simulink model "ARIES"  (R2024b)
settings: Solver=ode4  StartTime=0.0  StopTime=8*18601.8746  FixedStep=1e-1  RelTol=1e-3
model workspace (MAT data in the model file):
  BVH_bboxMax : Simulink.Parameter (value not decoded)
  BVH_bboxMin : Simulink.Parameter (value not decoded)
  BVH_fCount : Simulink.Parameter (value not decoded)
  BVH_fStart : Simulink.Parameter (value not decoded)
  BVH_faces : Simulink.Parameter (value not decoded)
  BVH_left : Simulink.Parameter (value not decoded)
  BVH_normals : Simulink.Parameter (value not decoded)
  BVH_right : Simulink.Parameter (value not decoded)
  BVH_vertexList : Simulink.Parameter (value not decoded)
  WP_NWaypoints : Simulink.Parameter (value not decoded)
  WP_STMArcs : Simulink.Parameter (value not decoded)
  WP_burnStrategy : Simulink.Parameter (value not decoded)
  WP_dtArc : Simulink.Parameter (value not decoded)
  WP_proxRadius : Simulink.Parameter (value not decoded)
  WP_waypointPosition : Simulink.Parameter (value not decoded)
  WP_waypointVelocity : Simulink.Parameter (value not decoded)
  asteroidAngularVelocity : Simulink.Parameter (value not decoded)
values from neighbouring files (symbols this model uses):
  actuators = actuatorsConfig()    [mainMontecarlo.m]    (also in mainSimulator.m)
  environment = environmentConfig(gravDataPath)    [mainMontecarlo.m]    (also in mainSimulator.m; mainWaypointGenerator.m = environmentConfig(gravDataPath, true))
  gravAtt = Simulink.Parameter(environment.gravStruct.gravAtt)    [mainSimulator.m]    (also in mainWaypointGenerator.m)
  init = initConditionConfig(control)    [mainMontecarlo.m]    (also in mainSimulator.m)
  simulation = simulationConfig()    [mainMontecarlo.m]    (also in mainSimulator.m = simulationConfig(control, environment))
symbols that are objects in the model workspace (value not decoded): asteroidAngularVelocity, BVH_bboxMax, BVH_bboxMin, BVH_faces, BVH_fCount, BVH_fStart, BVH_left, BVH_right, BVH_vertexList, WP_burnStrategy, WP_dtArc, WP_NWaypoints, WP_proxRadius, WP_STMArcs, WP_waypointPosition, WP_waypointVelocity
undefined symbols (not defined in the file or in its folder): control, magnitude, spacecraft
libraries: matrix_library x14, aerolibutil x4, sharedutil x2, sharedtransform x2, simulink x2
(part 2 of 2)

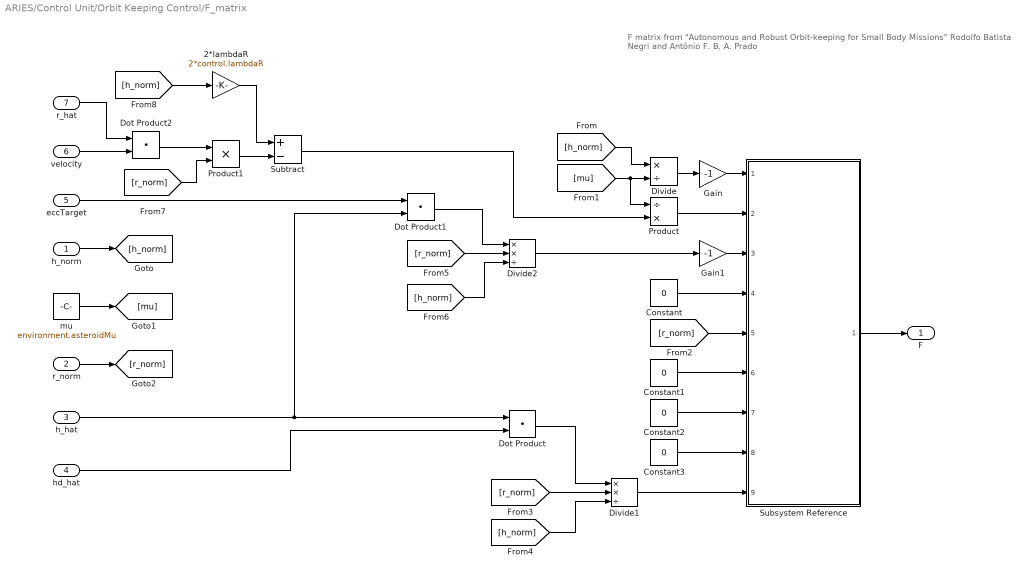
== system ARIES/Control Unit/Orbit Keeping Control/F_matrix ==
  note: F matrix from
      | "Autonomous and Robust Orbit-keeping for Small Body Missions"
      | Rodolfo Batista Negri and Antônio F. B. A. Prado
  h_norm : Inport
  r_norm : Inport  Port=2
  h_hat : Inport  Port=3
  hd_hat : Inport  Port=4
  eccTarget : Inport  Port=5
  velocity : Inport  Port=6
  r_hat : Inport  Port=7
  2*lambdaR : Gain  Gain=2*control.lambdaR
  Constant{,1..3} (4 alike) : Constant  Value=0
  Divide : Product  Inputs=*/
  Divide1 : Product  Inputs=**/
  Divide2 : Product  Inputs=**/
  Dot Product : DotProduct  OutDataTypeStr=Inherit: Inherit via internal rule
  Dot Product1 : DotProduct  OutDataTypeStr=Inherit: Inherit via internal rule
  Dot Product2 : DotProduct  OutDataTypeStr=Inherit: Inherit via internal rule
  Gain : Gain  Gain=-1
  Gain1 : Gain  Gain=-1
  Product : Product  Inputs=/*
  Product1 : Product  Inputs=**
  Subsystem Reference : Subsystem  ReferencedSubsystem=Create3x3Matrix
  Subtract : Sum  Inputs=+-
  mu : Constant  Value=environment.asteroidMu
  F : Outport
  wires:
  h_norm/1 -> [h_norm]
  mu/1 -> [mu]
  Subsystem Reference/1 -> F/1
  Divide/1 -> Gain/1
  [h_norm] -> Divide/1
  Gain/1 -> Subsystem Reference/1
  [mu] -> Product/1, Divide/2
  Constant/1 -> Subsystem Reference/4
  Constant1/1 -> Subsystem Reference/6
  Constant2/1 -> Subsystem Reference/7
  Constant3/1 -> Subsystem Reference/8
  r_norm/1 -> [r_norm]
  [r_norm] -> Subsystem Reference/5
  [r_norm] -> Divide1/2
  [h_norm] -> Divide1/3
  Dot Product/1 -> Divide1/1
  Divide1/1 -> Subsystem Reference/9
  h_hat/1 -> Dot Product1/2, Dot Product/1
  hd_hat/1 -> Dot Product/2
  eccTarget/1 -> Dot Product1/1
  Dot Product1/1 -> Divide2/1
  [h_norm] -> Divide2/3
  [r_norm] -> Divide2/2
  Divide2/1 -> Gain1/1
  Gain1/1 -> Subsystem Reference/3
  velocity/1 -> Dot Product2/2
  r_hat/1 -> Dot Product2/1
  Dot Product2/1 -> Product1/1
  [r_norm] -> Product1/2
  Product1/1 -> Subtract/2
  [h_norm] -> 2*lambdaR/1
  2*lambdaR/1 -> Subtract/1
  Subtract/1 -> Product/2
  Product/1 -> Subsystem Reference/2

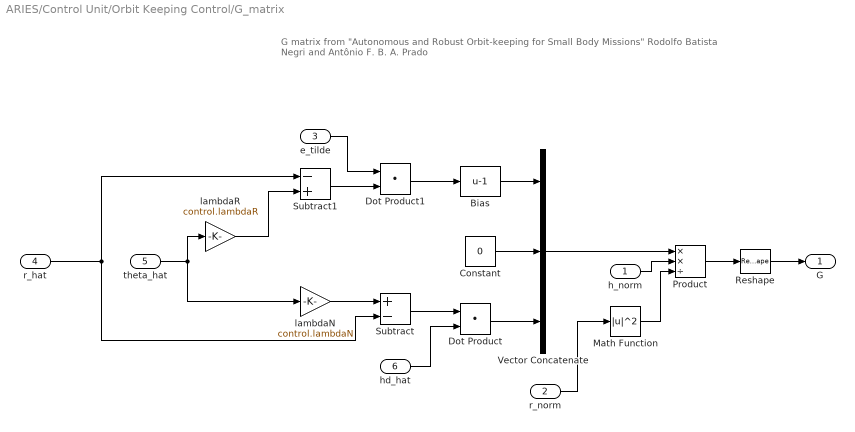
== system ARIES/Control Unit/Orbit Keeping Control/G_matrix ==
  note: G matrix from
      | "Autonomous and Robust Orbit-keeping for Small Body Missions"
      | Rodolfo Batista Negri and Antônio F. B. A. Prado
  h_norm : Inport
  r_norm : Inport  Port=2
  e_tilde : Inport  Port=3
  r_hat : Inport  Port=4
  theta_hat : Inport  Port=5
  hd_hat : Inport  Port=6
  Bias : Bias  Bias=-1  SaturateOnIntegerOverflow=off
  Constant : Constant  Value=0
  Dot Product : DotProduct  OutDataTypeStr=Inherit: Inherit via internal rule
  Dot Product1 : DotProduct  OutDataTypeStr=Inherit: Inherit via internal rule
  Math Function : Math  Operator=magnitude^2
  Product : Product  Inputs=**/
  Reshape : Reshape  OutputDimensionality=Column vector (2-D)
  Subtract : Sum  Inputs=+-
  Subtract1 : Sum  Inputs=-+
  Vector Concatenate : Concatenate  NumInputs=3
  lambdaN : Gain  Gain=control.lambdaN
  lambdaR : Gain  Gain=control.lambdaR
  G : Outport
  wires:
  Vector Concatenate/1 -> Product/1
  Constant/1 -> Vector Concatenate/2
  Product/1 -> Reshape/1
  h_norm/1 -> Product/2
  r_norm/1 -> Math Function/1
  Math Function/1 -> Product/3
  Dot Product/1 -> Vector Concatenate/3
  hd_hat/1 -> Dot Product/2
  lambdaN/1 -> Subtract/1
  theta_hat/1 -> lambdaN/1, lambdaR/1
  r_hat/1 -> Subtract/2, Subtract1/1
  Subtract/1 -> Dot Product/1
  Dot Product1/1 -> Bias/1
  e_tilde/1 -> Dot Product1/1
  Bias/1 -> Vector Concatenate/1
  Subtract1/1 -> Dot Product1/2
  lambdaR/1 -> Subtract1/2
  Reshape/1 -> G/1

== system ARIES/Control Unit/Orbit Keeping Control/f_RTN ==
  r_norm : Inport
  Constant1 : Constant  Value=environment.asteroidMu
  Constant2 : Constant  Value=[0;0]
  Divide : Product  Inputs=*/
  Gain : Gain  Gain=-1
  Math Function : Math  Operator=magnitude^2
  Reshape : Reshape  OutputDimensionality=Column vector (2-D)
  Vector Concatenate : Concatenate
  f_RTN : Outport
  wires:
  Divide/1 -> Gain/1
  Gain/1 -> Vector Concatenate/1
  r_norm/1 -> Math Function/1
  Math Function/1 -> Divide/2
  Constant1/1 -> Divide/1
  Vector Concatenate/1 -> Reshape/1
  Constant2/1 -> Vector Concatenate/2
  Reshape/1 -> f_RTN/1

== system ARIES/Control Unit/Orbit Keeping Control/||hys(s)||_inf ==
  s : Inport
  Max : MinMax  Function=max  Inputs=3
  Memory : Memory  InheritSampleTime=on
  Memory1 : Memory  InheritSampleTime=on
  Memory2 : Memory  InheritSampleTime=on
  Selector : Selector  InputPortWidth=3  IndexOptions=Index vector (dialog)  Indices=1  OutputSizes=1
  Selector1 : Selector  InputPortWidth=3  IndexOptions=Index vector (dialog)  Indices=2  OutputSizes=1
  Selector2 : Selector  InputPortWidth=3  IndexOptions=Index vector (dialog)  Indices=3  OutputSizes=1
  hys(s_1) : Subsystem  ReferencedSubsystem=hys_s
  hys(s_2) : Subsystem  ReferencedSubsystem=hys_s
  hys(s_3) : Subsystem  ReferencedSubsystem=hys_s
  ||hys(s)||_inf : Outport
  wires:
  hys(s_1)/1 -> Max/1, Memory/1
  Memory/1 -> hys(s_1)/1
  Memory1/1 -> hys(s_2)/1
  hys(s_2)/1 -> Memory1/1, Max/2
  hys(s_3)/1 -> Memory2/1, Max/3
  Memory2/1 -> hys(s_3)/1
  Selector/1 -> hys(s_1)/2
  s/1 -> Selector2/1, Selector/1, Selector1/1
  Selector1/1 -> hys(s_2)/2
  Selector2/1 -> hys(s_3)/2
  Max/1 -> ||hys(s)||_inf/1

== system ARIES/Control Unit/Waypoint guidance/Waypoint State Machine/gravAccel ==
  SCPosition : Inport  OutDataTypeStr=double  PortDimensions=3
  f : TriggerPort  TriggerType=function-call  VariantControl=(inherit)
      settings: CopyFcn=Stateflow.SLINSF.SimulinkMan.removeBlockPreDeleteFcn  PreDeleteFcn=Stateflow.SLINSF.SimulinkMan.unsafePredeleteFcn
  Constant : Constant  Value=[0:2]
  Constant1 : Constant  Value=[0 0 1]
  Gravitational Attraction interpolation with pre-lookup : Interpolation_n-D  NumberOfTableDimensions=4  Table=gravAtt  ExtrapMethod=Clip  InternalRulePriority=Speed  RndMeth=Simplest
      settings: InputPortMap=u0,u1,u2,u3,u4,u5,u6,u7
  Prelookup : PreLookup  BreakpointsData=environment.asteroidCoords.radius  BeginIndexSearchUsingPreviousIndexResult=on  ExtrapMethod=Linear  RndMeth=Simplest
  Prelookup1 : PreLookup  BreakpointsData=environment.asteroidCoords.polar  IndexSearchMethod=Linear search  BeginIndexSearchUsingPreviousIndexResult=on  DiagnosticForOutOfRangeInput=Warning  RndMeth=Simplest
  Prelookup2 : PreLookup  BreakpointsData=environment.asteroidCoords.azimuth  IndexSearchMethod=Linear search  BeginIndexSearchUsingPreviousIndexResult=on  RndMeth=Simplest
  cart2sphere : Subsystem  ReferencedSubsystem=cart2sphere
  gravAttraction : Outport
  wires:
  Constant1/1 -> Gravitational Attraction interpolation with pre-lookup/8
  Prelookup/2 -> Gravitational Attraction interpolation with pre-lookup/2
  cart2sphere/3 -> Prelookup2/1
  Prelookup1/2 -> Gravitational Attraction interpolation with pre-lookup/4
  cart2sphere/1 -> Prelookup/1
  Constant/1 -> Gravitational Attraction interpolation with pre-lookup/7
  Prelookup2/2 -> Gravitational Attraction interpolation with pre-lookup/6
  Prelookup1/1 -> Gravitational Attraction interpolation with pre-lookup/3
  Prelookup/1 -> Gravitational Attraction interpolation with pre-lookup/1
  cart2sphere/2 -> Prelookup1/1
  Prelookup2/1 -> Gravitational Attraction interpolation with pre-lookup/5
  SCPosition/1 -> cart2sphere/1
  Gravitational Attraction interpolation with pre-lookup/1 -> gravAttraction/1

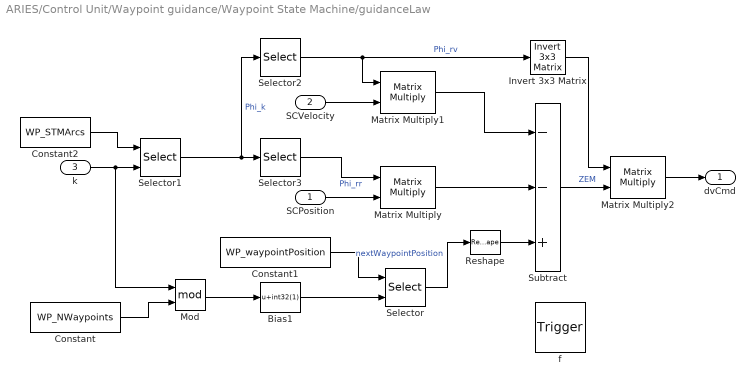
== system ARIES/Control Unit/Waypoint guidance/Waypoint State Machine/guidanceLaw ==
  SCPosition : Inport  OutDataTypeStr=double  PortDimensions=3
  SCVelocity : Inport  Port=2  OutDataTypeStr=double  PortDimensions=3
  k : Inport  Port=3  OutDataTypeStr=int32  PortDimensions=1
  f : TriggerPort  TriggerType=function-call  VariantControl=(inherit)
      settings: CopyFcn=Stateflow.SLINSF.SimulinkMan.removeBlockPreDeleteFcn  PreDeleteFcn=Stateflow.SLINSF.SimulinkMan.unsafePredeleteFcn
  Bias1 : Bias  Bias=int32(1)  SaturateOnIntegerOverflow=off
  Constant : Constant  Value=WP_NWaypoints
  Constant1 : Constant  Value=WP_waypointPosition
  Constant2 : Constant  Value=WP_STMArcs
  Invert 3x3 Matrix : aerolibutil/Invert  3x3 Matrix
  Matrix Multiply : Product  Multiplication=Matrix(*)
  Matrix Multiply1 : Product  Multiplication=Matrix(*)
  Matrix Multiply2 : Product  Multiplication=Matrix(*)
  Mod : Math  Operator=mod
  Reshape : Reshape
  Selector : Selector  NumberOfDimensions=2  InputPortWidth=3  IndexOptions=Index vector (port),Select all  Indices=[1 3],1  OutputSizes=1,1
  Selector1 : Selector  NumberOfDimensions=3  InputPortWidth=3  IndexOptions=Select all,Select all,Index vector (port)  Indices=[1 3],1,1  OutputSizes=1,1,1
  Selector2 : Selector  NumberOfDimensions=2  InputPortWidth=3  IndexOptions=Index vector (dialog),Index vector (dialog)  Indices=1:3,4:6  OutputSizes=1,1
  Selector3 : Selector  NumberOfDimensions=2  InputPortWidth=3  IndexOptions=Index vector (dialog),Index vector (dialog)  Indices=1:3,1:3  OutputSizes=1,1
  Subtract : Sum  Inputs=--+
  dvCmd : Outport  OutputWhenDisabled=reset  InitialOutput=zeros(3,1)
  wires:
  Mod/1 -> Bias1/1
  Constant2/1 -> Selector1/1
  Selector2/1 -> Matrix Multiply1/1, Invert 3x3 Matrix/1  "Phi_rv"
  k/1 -> Selector1/2, Mod/1
  Constant/1 -> Mod/2
  SCVelocity/1 -> Matrix Multiply1/2
  Selector3/1 -> Matrix Multiply/1  "Phi_rr"
  SCPosition/1 -> Matrix Multiply/2
  Constant1/1 -> Selector/1
  Bias1/1 -> Selector/2
  Matrix Multiply1/1 -> Subtract/1
  Matrix Multiply/1 -> Subtract/2
  Selector/1 -> Reshape/1  "nextWaypointPosition"
  Invert 3x3 Matrix/1 -> Matrix Multiply2/1
  Subtract/1 -> Matrix Multiply2/2  "ZEM"
  Matrix Multiply2/1 -> dvCmd/1
  Reshape/1 -> Subtract/3
  Selector1/1 -> Selector2/1, Selector3/1  "Phi_k"

== system ARIES/Control Unit/Waypoint guidance/Waypoint State Machine/nearWaypoint ==
  SCPosition : Inport  OutDataTypeStr=double  PortDimensions=3
  k : Inport  Port=2  OutDataTypeStr=int32  PortDimensions=1
  f : TriggerPort  TriggerType=function-call  VariantControl=(inherit)
      settings: CopyFcn=Stateflow.SLINSF.SimulinkMan.removeBlockPreDeleteFcn  PreDeleteFcn=Stateflow.SLINSF.SimulinkMan.unsafePredeleteFcn
  Constant : Constant  Value=WP_waypointPosition
  Constant2 : Constant  Value=WP_proxRadius
  LessThanOrEqual : RelationalOperator  Operator=<=  OutDataTypeStr=boolean  RndMeth=Simplest  InputSameDT=off
  Reshape : Reshape
  Selector : Selector  NumberOfDimensions=2  InputPortWidth=[WP_NWaypoints 3]  IndexOptions=Index vector (port),Select all  Indices=[1 3],1  OutputSizes=1,1
  Subsystem Reference : Subsystem  ReferencedSubsystem=VectorNorm
  Subtract : Sum  Inputs=+-
  res : Outport  OutputWhenDisabled=reset  InitialOutput=false
  wires:
  Reshape/1 -> Subtract/2
  Constant/1 -> Selector/1
  Subsystem Reference/1 -> LessThanOrEqual/1
  k/1 -> Selector/2
  Selector/1 -> Reshape/1
  SCPosition/1 -> Subtract/1
  Subtract/1 -> Subsystem Reference/1
  Constant2/1 -> LessThanOrEqual/2
  LessThanOrEqual/1 -> res/1

== system ARIES/External Environment/Accelerations/2BPGravity ==
  r : Inport
  Divide : Product  Inputs=*/*
  Gain : Gain  Gain=-1
  Power : Math  Operator=pow
  VectorNorm : Subsystem  ReferencedSubsystem=VectorNorm
  cube : Constant  Value=3
  mu_sun : Constant  Value=environment.mu_sun
  2BPAcc : Outport
  wires:
  mu_sun/1 -> Gain/1
  Divide/1 -> 2BPAcc/1
  Gain/1 -> Divide/3
  r/1 -> Divide/1, VectorNorm/1
  VectorNorm/1 -> Power/1
  Power/1 -> Divide/2
  cube/1 -> Power/2

== system ARIES/External Environment/Accelerations/3BPSun ==
  SCPosition : Inport
  C_BI : Inport  Port=2
  AsteroidPosition : Inport  Port=3
  Add : Sum
  Constant : Constant  Value=3
  Constant1 : Constant  Value=3
  Divide : Product  Inputs=*/
  Divide1 : Product  Inputs=*/
  Gain : Gain  Gain=-1
  Matrix Multiply : Product  Multiplication=Matrix(*)
  Power : Math  Operator=pow
  Power1 : Math  Operator=pow
  Product : Product
  Subtract : Sum  Inputs=+-
  TBP Acceleartion : ToWorkspace  Commented=on  VariableName=TBPAcc  SaveFormat=Timeseries  SampleTime=-1
  mu_sun : Constant  Value=environment.mu_sun
  || (r_B)_B + (r_S)_B || : Subsystem  ReferencedSubsystem=VectorNorm
  || r_B || : Subsystem  ReferencedSubsystem=VectorNorm
  3BPAcc : Outport
  wires:
  mu_sun/1 -> Gain/1
  Gain/1 -> Product/2
  Product/1 -> TBP Acceleartion/1, 3BPAcc/1
  AsteroidPosition/1 -> Matrix Multiply/2  "(r_B)_I"
  C_BI/1 -> Matrix Multiply/1
  Matrix Multiply/1 -> Add/2, Divide/1, || r_B ||/1  "(r_B)_B"
  Subtract/1 -> Product/1
  || r_B ||/1 -> Power/1
  Constant/1 -> Power/2
  Power/1 -> Divide/2
  Divide/1 -> Subtract/2
  SCPosition/1 -> Add/1  "(r_S)_B"
  Power1/1 -> Divide1/2
  Constant1/1 -> Power1/2
  || (r_B)_B + (r_S)_B ||/1 -> Power1/1
  Add/1 -> || (r_B)_B + (r_S)_B ||/1, Divide1/1  "(r_B)_B + (r_S)_B"
  Divide1/1 -> Subtract/1

== system ARIES/External Environment/Accelerations/EulerEquation ==
  note: External torques
      | in F_S
  note: Input
  w_s : Inport
  SRPTau : Inport  Port=2
  Bus Element In3 : Inport  Port=3  PortName=actuatorsBus  Element=rw.hr
  Bus Element In1 : Inport  Port=3  PortName=actuatorsBus  Element=rw.dhr
  Bus Element In2 : Inport  Port=3  PortName=actuatorsBus  Element=attThruster.tauDesat
  Add : Sum
  Constant : Constant  Value=spacecraft.I_inv
  Constant1 : Constant  Value=spacecraft.I_mat
  Cross Product : matrix_library/Cross Product
  Matrix Multiply : Product  Multiplication=Matrix(*)
  Matrix Multiply2 : Product  Multiplication=Matrix(*)
  Sum : Sum  Inputs=+--+
  dw : Outport
  wires:
  w_s/1 -> [ws]
  [ws] -> Cross Product/1
  Constant/1 -> Matrix Multiply/1
  Constant1/1 -> Matrix Multiply2/1
  [ws] -> Matrix Multiply2/2
  Matrix Multiply2/1 -> Add/1  "I * w"
  SRPTau/1 -> Sum/1
  Cross Product/1 -> Sum/2  "w x (Iw)"
  Sum/1 -> Matrix Multiply/2
  Matrix Multiply/1 -> dw/1  "dot(w) in F_S"
  Add/1 -> Cross Product/2
  Bus Element In3/1 -> Add/2
  Bus Element In1/1 -> Sum/3
  Bus Element In2/1 -> Sum/4

== system ARIES/External Environment/Accelerations/Fictious ==
  SCPosition : Inport
  SCVelocity : Inport  Port=2
  AsteroidAngVelocity : Inport  Port=3
  Add : Sum  Inputs=--
  Cross Product : matrix_library/Cross Product
  Cross Product1 : matrix_library/Cross Product
  Cross Product2 : matrix_library/Cross Product
  Fictious Acceleartions : ToWorkspace  Commented=on  VariableName=FictiousAcc  SaveFormat=Timeseries  SampleTime=-1
  Gain : Gain  Gain=2
  CoriolisCentrifugalAcc : Outport
  wires:
  AsteroidAngVelocity/1 -> Cross Product1/1, Cross Product/1, Cross Product2/1
  Cross Product1/1 -> Cross Product2/2
  SCPosition/1 -> Cross Product1/2
  Add/1 -> Fictious Acceleartions/1, CoriolisCentrifugalAcc/1
  SCVelocity/1 -> Cross Product/2
  Cross Product/1 -> Gain/1
  Cross Product2/1 -> Add/1
  Gain/1 -> Add/2

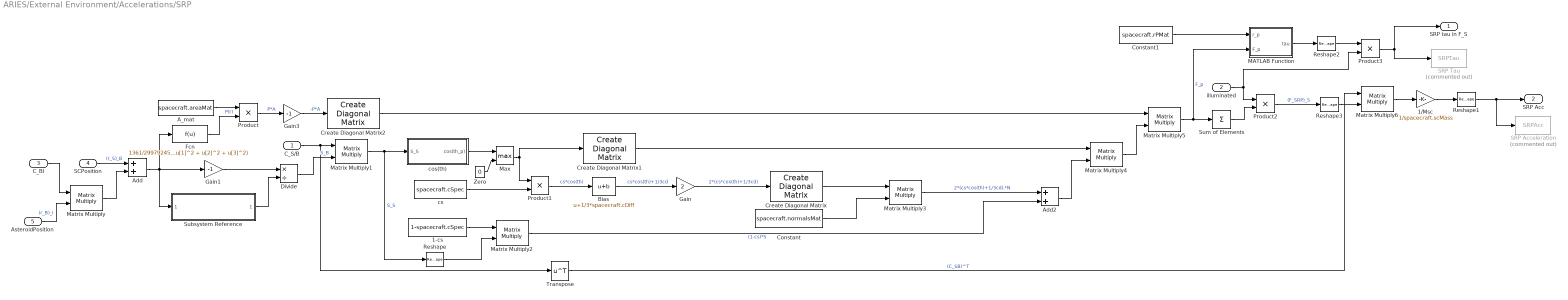
== system ARIES/External Environment/Accelerations/SRP ==
  C_S/B : Inport
  illuminated : Inport  Port=2
  C_BI : Inport  Port=3
  SCPosition : Inport  Port=4
  AsteroidPosition : Inport  Port=5
  1-cs : Constant  Value=1-spacecraft.cSpec
  1/Msc : Gain  Gain=1/spacecraft.scMass
  A_mat : Constant  Value=spacecraft.areaMat
  Add : Sum
  Add2 : Sum
  Bias : Bias  Bias=1/3*spacecraft.cDiff  SaturateOnIntegerOverflow=off
  Constant : Constant  Value=spacecraft.normalsMat
  Constant1 : Constant  Value=spacecraft.rPMat
  Create Diagonal Matrix : matrix_library/Create Diagonal Matrix
      settings: LibrarySourceBlock=|
      | simulink/Matrix
      | Operations/Create Diagonal
      | Matrix
  Create Diagonal Matrix1 : matrix_library/Create Diagonal Matrix
      settings: LibrarySourceBlock=|
      | simulink/Matrix
      | Operations/Create Diagonal
      | Matrix
  Create Diagonal Matrix2 : matrix_library/Create Diagonal Matrix
      settings: LibrarySourceBlock=|
      | simulink/Matrix
      | Operations/Create Diagonal
      | Matrix
  Divide : Product  Inputs=*/
  Fcn : Fcn  Expr=1361/299792458 * (149598000*1e3)^2 / (u[1]^2 + u[2]^2 + u[3]^2)
  Gain : Gain  Gain=2
  Gain1 : Gain  Gain=-1
  Gain3 : Gain  Gain=-1
  MATLAB Function : MATLAB Function  TreatAsAtomicUnit=on
  Matrix Multiply{,1..6} (7 alike) : Product  Multiplication=Matrix(*)
  Max : MinMax  Function=max  Inputs=2
  Product{,1..3} (4 alike) : Product
  Reshape : Reshape  OutputDimensionality=Row vector (2-D)
  Reshape1 : Reshape
  Reshape2 : Reshape
  Reshape3 : Reshape
  SRP Acceleration : ToWorkspace  Commented=on  VariableName=SRPAcc  SaveFormat=Timeseries  SampleTime=-1
  SRP Tau : ToWorkspace  Commented=on  VariableName=SRPTau  SaveFormat=Timeseries  SampleTime=-1
  Subsystem Reference : Subsystem  ReferencedSubsystem=VectorNorm
  Sum of Elements : Sum  Inputs=+  CollapseMode=Specified dimension
  Transpose : Math  Operator=transpose
  Zero : Constant  Value=0  OutDataTypeStr=Inherit: Inherit via back propagation
  cos(th) : Subsystem
  cs : Constant  Value=spacecraft.cSpec
  SRP tau in F_S : Outport
  SRP Acc : Outport  Port=2
  wires:
  illuminated/1 -> Product3/2, Product2/1
  Divide/1 -> Matrix Multiply1/2  "S_B"
  SCPosition/1 -> Add/1  "(r_S)_B"
  C_BI/1 -> Matrix Multiply/1
  AsteroidPosition/1 -> Matrix Multiply/2  "(r_B)_I"
  Fcn/1 -> Product/2  "P(r)"
  Matrix Multiply/1 -> Add/2
  A_mat/1 -> Product/1
  Product/1 -> Gain3/1  "P*A"
  Create Diagonal Matrix1/1 -> Matrix Multiply4/1
  Matrix Multiply2/1 -> Add2/2  "(1-cs)*S"
  Add/1 -> Fcn/1, Gain1/1, Subsystem Reference/1
  Create Diagonal Matrix2/1 -> Matrix Multiply5/1
  Gain3/1 -> Create Diagonal Matrix2/1  "-P*A"
  Subsystem Reference/1 -> Divide/2
  Create Diagonal Matrix/1 -> Matrix Multiply3/1
  Product1/1 -> Bias/1  "cs*cos(th)"
  C_S/B/1 -> Transpose/1, Matrix Multiply1/1
  Matrix Multiply1/1 -> cos(th)/1(S_S), Reshape/1  "S_S"
  cos(th)/1(cos(th_p)) -> Max/1
  cs/1 -> Product1/2
  Matrix Multiply6/1 -> 1/Msc/1
  1-cs/1 -> Matrix Multiply2/1
  Reshape/1 -> Matrix Multiply2/2
  Bias/1 -> Gain/1  "cs*cos(th)+1/3cd"
  Transpose/1 -> Matrix Multiply6/1  "(C_SB)^T"
  Gain/1 -> Create Diagonal Matrix/1  "2*(cs*cos(th)+1/3cd)"
  Constant/1 -> Matrix Multiply3/2
  Matrix Multiply3/1 -> Add2/1  "2*(cs*cos(th)+1/3cd).*N"
  Add2/1 -> Matrix Multiply4/2
  Matrix Multiply4/1 -> Matrix Multiply5/2
  Sum of Elements/1 -> Product2/2
  1/Msc/1 -> Reshape1/1
  Reshape1/1 -> SRP Acc/1, SRP Acceleration/1
  Max/1 -> Create Diagonal Matrix1/1, Product1/1
  Zero/1 -> Max/2
  Product2/1 -> Reshape3/1  "(F_SRP)_S"
  Constant1/1 -> MATLAB Function/1(r_p)
  Matrix Multiply5/1 -> MATLAB Function/2(F_p), Sum of Elements/1  "F_p"
  MATLAB Function/1(tau) -> Reshape2/1
  Product3/1 -> SRP tau in F_S/1, SRP Tau/1
  Reshape2/1 -> Product3/1
  Gain1/1 -> Divide/1
  Reshape3/1 -> Matrix Multiply6/2

== system ARIES/External Environment/Accelerations/stopConditionComputation ==
  gravLaplace : Inport
  Abs : Abs  SaturateOnIntegerOverflow=off
  Add Constant : Bias  Bias=-4*pi  SaturateOnIntegerOverflow=off
  Constant2 : Constant  Value=environment.gravLaplaceTol
  Less Than : RelationalOperator  Operator=<  OutDataTypeStr=boolean  RndMeth=Simplest  InputSameDT=off
  StopCondition : Outport
  wires:
  Constant2/1 -> Less Than/2
  gravLaplace/1 -> Add Constant/1
  Abs/1 -> Less Than/1
  Add Constant/1 -> Abs/1
  Less Than/1 -> StopCondition/1

== system ARIES/External Environment/DerivativeStateAssembly/dq//dt ==
  q_SB : Inport
  C_S/B : Inport  Port=2
  SCAngVel : Inport  Port=3
  Constant : Constant  Value=environment.asteroidAngularVelocity
  Gain4 : Gain  Gain=0.5
  Matrix Multiply : Product  Multiplication=Matrix(*)
  Quaternion Multiplication : aerolibutil/Quaternion Multiplication
  Sum : Sum  Inputs=|+-
  Vector Concatenate : Concatenate
  Zero : Constant  Value=0  OutDataTypeStr=Inherit: Inherit via back propagation
  dQ : Outport
  wires:
  Quaternion Multiplication/1 -> Gain4/1
  q_SB/1 -> Quaternion Multiplication/2
  Gain4/1 -> dQ/1
  Constant/1 -> Matrix Multiply/2
  SCAngVel/1 -> Sum/1
  Sum/1 -> Vector Concatenate/2  "w_rel"
  Zero/1 -> Vector Concatenate/1
  Vector Concatenate/1 -> Quaternion Multiplication/1
  C_S/B/1 -> Matrix Multiply/1
  Matrix Multiply/1 -> Sum/2

== system ARIES/External Environment/OrbitCounter/Triggered Subsystem ==
  In1 : Inport
  Trigger : TriggerPort  VariantControl=(inherit)
  Add Constant : Bias  Bias=1  SaturateOnIntegerOverflow=off
  Out1 : Outport  InitialOutput=0
  wires:
  In1/1 -> Add Constant/1
  Add Constant/1 -> Out1/1

== system ARIES/Actuators/Reaction wheels + thrusters/tauDesatComputation/If Action Subsystem ==
  Action Port : ActionPort  ActionPortLabel=if(u1 == 1 & u2 == 1)
  Zero : Constant  Value=0  OutDataTypeStr=Inherit: Inherit via back propagation
  Out1 : Outport
  wires:
  Zero/1 -> Out1/1

== system ARIES/Actuators/Reaction wheels + thrusters/tauDesatComputation/If Action Subsystem1 ==
  Action Port : ActionPort  ActionPortLabel=elseif(u1 == 0 & u3 == 1)
  Zero : Constant  OutDataTypeStr=Inherit: Inherit via back propagation
  Out1 : Outport
  wires:
  Zero/1 -> Out1/1

== system ARIES/Actuators/Reaction wheels + thrusters/tauDesatComputation/If Action Subsystem2 ==
  In1 : Inport
  Action Port : ActionPort  ActionPortLabel=else
  Out1 : Outport
  wires:
  In1/1 -> Out1/1

== system ARIES/Attitude Control/Variant Subsystem/ZENITH/sign correction ==
  q_in : Inport
  Gain : Gain  Gain=-1
  Selector : Selector  InputPortWidth=4  IndexOptions=Index vector (dialog)  Indices=1  OutputSizes=1
  Switch : Switch  Criteria=u2 > Threshold  SaturateOnIntegerOverflow=off  InputSameDT=off
  q_out : Outport
  wires:
  q_in/1 -> Gain/1, Switch/1, Selector/1
  Selector/1 -> Switch/2
  Switch/1 -> q_out/1
  Gain/1 -> Switch/3

== system ARIES/External Environment/Accelerations/SRP/cos(th) ==
  S_S : Inport
  Constant : Constant  Value=spacecraft.normalsMat(:,1)
  Constant1 : Constant  Value=spacecraft.normalsMat(:,2)
  Constant2 : Constant  Value=spacecraft.normalsMat(:,3)
  Product : Product
  Product1 : Product
  Product2 : Product
  Selector : Selector  InputPortWidth=3  IndexOptions=Index vector (dialog)  Indices=1  OutputSizes=1
  Selector1 : Selector  InputPortWidth=3  IndexOptions=Index vector (dialog)  Indices=2  OutputSizes=1
  Selector2 : Selector  InputPortWidth=3  IndexOptions=Index vector (dialog)  Indices=3  OutputSizes=1
  Sum of Elements : Sum  Inputs=+  CollapseMode=Specified dimension  CollapseDim=2
  Vector Concatenate : Concatenate  NumInputs=3  Mode=Multidimensional array  ConcatenateDimension=2
  cos(th_p) : Outport
  wires:
  S_S/1 -> Selector/1, Selector1/1, Selector2/1
  Selector/1 -> Product/1
  Vector Concatenate/1 -> Sum of Elements/1
  Product1/1 -> Vector Concatenate/2
  Product/1 -> Vector Concatenate/1
  Selector2/1 -> Product2/1
  Constant1/1 -> Product1/2
  Constant/1 -> Product/2
  Selector1/1 -> Product1/1
  Constant2/1 -> Product2/2
  Product2/1 -> Vector Concatenate/3
  Sum of Elements/1 -> cos(th_p)/1  "sum(S.*N,2)"

== matlab function ARIES/External Environment/Accelerations/SRP/MATLAB Function ==
  data: r_p input; F_p input; tau output
function tau = fcn(r_p, F_p)
    %#codegen
    tau = sum(cross(r_p, F_p),1);

== matlab function ARIES/Distance And Shadow/pointToMeshDistanceAndShadow ==
  data: position input; sunDir input; BVH_bboxMin parameter; BVH_bboxMax parameter; BVH_left parameter; BVH_right parameter; BVH_fStart parameter; BVH_fCount parameter; dist output; BVH_vertexList parameter; illuminated output; BVH_faces parameter
function [dist, illuminated] = pointToMeshDistanceAndShadow(position, sunDir, BVH_bboxMin, BVH_bboxMax, BVH_left, ...
        BVH_right, BVH_fStart, BVH_fCount, BVH_vertexList, BVH_faces)

    % position: [3x1] satellite's position
    % sunDir: [3x1] Normalized Sun direction FROM spacecraft TO Sun

    %#codegen

    % persistent lastLeafDist lastOccTri
    % 
    % if isempty(lastLeafDist) || isempty(lastOccTri)
    %     lastLeafDist = int32(1);    % Last leaf for which minimum distance was found
    %     lastOccTri   = int32(0);    % Last triangle that occluded sunlight
    % end

    % Origin for shadow computation (slight offset to avoid
    % self-intersection)
    rayOrigin = position + 1e-9*sunDir;

    % Initialize minimum distance found and shadow check
    dmin2 = Inf;
    inShadow = false;

    

    %% Dual cache predictor

    % numFaces = int32(size(BVH_faces,1));
    % 
    % % Cached shadow triangle
    % if (lastOccTri > 0) && (lastOccTri <= numFaces)
    %     faceIdx = BVH_faces(lastOccTri, :);
    %     if rayTriangleIntersection(rayOrigin, sunDir, BVH_vertexList(faceIdx(1), :), ...
    %             BVH_vertexList(faceIdx(2), :), BVH_vertexList(faceIdx(3), :))
    %         inShadow = true;
    %     end
    % end
    % 
    % % Cached distance leaf
    % if BVH_left(lastLeafDist) == -1
    %     % Index in faces array where this leaf's faces begin
    %     fStartIdx = BVH_fStart(lastLeafDist);
    %     % Number of faces in this leaf
    %     faceNum = BVH_fCount(lastLeafDist);
    % 
    %     for ii = int32(0):faceNum-1
    %         faceIdx = BVH_faces(fStartIdx+ii, :);
    %         dFace2 = distPointTriangleSquared(rayOrigin, BVH_vertexList(faceIdx(1), :), ...
    %                 BVH_vertexList(faceIdx(2), :), BVH_vertexList(faceIdx(3), :));
    %         if dFace2 < dmin2
    %             dmin2 = dFace2;
    %         end
    %     end
    % end

    %% BVH Traversal

    MAX_STACK = int32(256);
    stack = zeros(MAX_STACK, 1, 'int32');
    stackPointer = int32(1);

    % Set stack root
    stack(stackPointer) = int32(1);

    % bestLeaf = lastLeafDist;

    while stackPointer > 0
        currentNode = stack(stackPointer);
        stackPointer = stackPointer - 1;

        dBox2 = distPointAABBoxSquared(position, BVH_bboxMin(currentNode, :), BVH_bboxMax(currentNode, :));

        rayHit = rayAABBIntersection(rayOrigin, sunDir, BVH_bboxMin(currentNode, :), BVH_bboxMax(currentNode, :));

        if (dBox2 >= dmin2) && ~rayHit
            continue
        end

        % Check if we have a leaf or if there are children nodes
        if BVH_left(currentNode) == -1
            % Index in faces array where this leaf's faces begin
            fStartIdx = BVH_fStart(currentNode);
            % Number of faces in this leaf
            faceNum = BVH_fCount(currentNode);
            
            for ii = int32(0):faceNum-1
                faceIdx = BVH_faces(fStartIdx+ii, :);
                vertA = BVH_vertexList(faceIdx(1), :);
                vertB = BVH_vertexList(faceIdx(2), :);
                vertC = BVH_vertexList(faceIdx(3), :);
                
                % Distance from face
                dFace2 = distPointTriangleSquared(position, vertA, vertB, vertC);
                if dFace2 < dmin2
                    dmin2 = dFace2;
                    % bestLeaf = currentNode;
                end
                
                % Shadow detection
                if ~inShadow
                    if rayTriangleIntersection(rayOrigin, sunDir, vertA, vertB, vertC)
                        inShadow = true;
                        % lastOccTri = fStartIdx+ii;
                    end
                end

            end
        else
            
            % Distance-ordered traversal
            leftNode = BVH_left(currentNode);
            rightNode = BVH_right(currentNode);

            dLeft2 = distPointAABBoxSquared(position, BVH_bboxMin(leftNode, :), BVH_bboxMax(leftNode, :));
            dRight2 = distPointAABBoxSquared(position, BVH_bboxMin(rightNode, :), BVH_bboxMax(rightNode, :));

            % Stack is LIFO so last node inserted is the first one to be
            % processed
            if dLeft2 < dRight2
                stackPointer = stackPointer + 1;
                stack(stackPointer) = rightNode;
                stackPointer = stackPointer + 1;
                stack(stackPointer) = leftNode;
            else
                stackPointer = stackPointer + 1;
                stack(stackPointer) = leftNode;
                stackPointer = stackPointer + 1;
                stack(stackPointer) = rightNode;
            end


        end
    end

    % lastLeafDist = bestLeaf;
    dist = sqrt(dmin2);
    illuminated = ~inShadow;
    
end

function distSq = distPointAABBoxSquared(position, bboxMin, bboxMax)
    % Implemented from 
    % Christer Ericson, “Real-Time Collision Detection” (pp. 132)

    %#codegen
    distSq = 0;
    for ii = 1:3
        if position(ii) < bboxMin(ii)
            t = bboxMin(ii) - position(ii);
        elseif position(ii) > bboxMax(ii)
            t = position(ii) - bboxMax(ii);
        else
            t = 0;
        end
        distSq = distSq + t*t;
    end
end

function dist = distPointTriangle(position, vertA, vertB, vertC)
    % Implemented from 
    % Christer Ericson, “Real-Time Collision Detection” (pp. 136-142)
    % Reference pseudo-code at pp. 141-142

    %#codegen
    AB = vertB - vertA;
    AC = vertC - vertA;
    AP = position - vertA;
    
    % Check if P is in the vertex region outside A
    d1 = dot(AB, AP); % Projection of AP on AB
    d2 = dot(AC, AP);

    % If the projection of AP on both AB and AC is negative it means that
    % A is closest vertex to P, so the distance from the face is AP
    % In terms of barycentric coordinates: (1,0,0)
    if d1 <= 0 && d2 <= 0
        dist = norm(AP);
        return
    end

    % Check if P is in the vertex region outside B
    BP = position - vertB;
    d3 = dot(AB, BP);
    d4 = dot(AC, BP); 

    % If the point P is beyond B and not closer to BC or the face, then
    % B is closest vertex to P, so the distance from the face is BP
    % In terms of barycentric coordinates: (0,1,0)
    if d3 >= 0 && d4 <= d3
        dist = norm(BP);
        return
    end

    % Check if P is in the vertex region outside B
    CP = position - vertC;
    d5 = dot(AB, CP);
    d6 = dot(AC, CP);

    % If the point P is beyond C and not closer to BC or the face, then
    % C is closest vertex to P, so the distance from the face is CP
    % In terms of barycentric coordinates: (0,0,1)
    if d6 >= 0 && d5 <= d6
        dist = norm(CP);
        return
    end

    % Check if P is in the edge region of AB, if so distance is computed
    % between P and its projection onto AB
    vc = d1*d4 - d3*d2;

    if vc <= 0 && d1 >= 0 && d3 <= 0
        v = d1/(d1 - d3);
        proj = vertA + v * AB; % Barycentric coordinates (1-v,v,0)
        dist = norm(position - proj);
        return
    end

    % Check if P is in the edge region of AC, if so distance is computed
    % between P and its projection onto AC
    vb = d5*d2 - d1*d6;

    if vb <= 0 && d2 >= 0 && d6 <= 0
        w = d2 / (d2 - d6);
        proj = vertA + w * AC; % Barycentric coordinates (1-w,0,w)
        dist = norm(position - proj);
        return 
    end

    % Check if P is in the edge region of BC, if so distance is computed
    % between P and its projection onto BC
    va = d3*d6 - d5*d4;
    if va <= 0 && (d4 - d3) >= 0 && (d5 - d6) >= 0
        w = (d4 - d3)/((d4 - d3) + (d5 - d6));
        proj = vertB + w * (vertC - vertB); % Barycentric coordinates (0,1-w,w)
        dist = norm(position - proj);
        return
    end

    % If all previous checks failed it means P is inside the face region.
    % Compute the face normal and the distance of P from a vertex of the
    % triangle along such normal
    % Note: This is different from the pseudo-code at pp.141-142 of 
    % Christer Ericson, “Real-Time Collision Detection” as the barycentric
    % coordinates are not needed, thus the projection is computed
    % "implicitely"
    normal = cross(AB, AC); normal = normal/norm(normal);
    dist = abs(dot(position-vertA, normal));

end

function dist2 = distPointTriangleSquared(position, vertA, vertB, vertC)
    %#codegen
    dist = distPointTriangle(position, vertA, vertB, vertC);
    dist2 = dist*dist;
end

function rayHit = rayAABBIntersection(rayOrigin, rayDir, bboxMin, bboxMax)
    % Slab method implemented from
    % Kay, Timothy L.; Kajiya, James T., "Ray Tracing Complex Scenes"
    %#codegen

    epsVal = 1e-12; % Minimum value below which ray is considered parallel to edge

    tClose = -Inf; tFar = Inf;

    for ii = 1:3
        if abs(rayDir) < epsVal
            if rayOrigin(ii) < bboxMin(ii) || rayOrigin(ii) > bboxMax(ii)
                rayHit = false;
                return
            end
        else
            tLow = (bboxMin(ii) - rayOrigin(ii))/rayDir(ii);
            tHigh = (bboxMax(ii) - rayOrigin(ii))/rayDir(ii);

            tClose = max(tClose, min(tLow, tHigh));
            tFar = min(tFar, max(tLow, tHigh));

            if tClose > tFar 
                rayHit = false;
                return
            end
        end
    end
    
    rayHit = (tFar>0);
end

function rayHit = rayTriangleIntersection(rayOrigin, rayDir, vertA, vertB, vertC)
    % Implemented from 
    % Tomas Moller, Ben Trumbore, "Fast Minimum Storage Ray/Triangle Intersection"

    %#codegen
    
    epsVal = 1e-12; % Minimum value below which ray is considered parallel to triangle

    edge1 = vertB - vertA;
    edge2 = vertC - vertA;
    
    pVec = cross(rayDir, edge2);
    det = dot(edge1, pVec);

    % If determinant is near zero, ray lies in the plane of the triangle
    if abs(det) < epsVal
        rayHit = false;
        return
    end

    tVec = rayOrigin - vertA;
    u = dot(tVec, pVec)/det;
    if u < 0 || u > 1
       rayHit = false;
       return
    end

    qVec = cross(tVec, edge1);
    v = dot(rayDir, qVec)/det;
    if v < 0 || (u + v) > 1
        rayHit = false;
        return
    end

    t = dot(edge2, qVec)/det;
    rayHit = (t > epsVal);
end

== matlab function ARIES/Attitude Control/Attitude error DCM/MATLAB Function ==
  data: Ae_vec output; Ce input
function Ae_vec = AttErrVec(Ce)
    %#codegen

    if trace(Ce) < -0.5
        % Extract rotation axis
        CeI = Ce + eye(3);
        [~, idx] = max(diag(CeI)); % Find largest diagonal element
        n = CeI(:, idx);
        n = n / norm(n);
        if n(idx) < 0
            n = -n;
        end
        Ae_vec = pi*n;
    else
        Ae = Ce - Ce';
        Ae_vec = [Ae(3,2); Ae(1,3); Ae(2,1)];
    end

end

== stateflow chart ARIES/Control Unit/Waypoint guidance/Waypoint State Machine ==
  state ACTIVE_BURN
    state SINGLE_BURN
      entry:
      burnActive = true;
      during:
      controlAcc = dvCmd / tBurn;
      stepsLeft = stepsLeft - int32(1);
      currentWpIdx = k;
    state TWO_STAGE
      state ARRIVAL_BURN
        entry:
        burnActive = true
        during:
        controlAcc = dvArr / tBurn;
        stepsArrLeft = stepsArrLeft - int32(1);
      state INTER_BURN_COOLDOWN
        entry:
        controlAcc = zeros(3,1);
        burnActive = false;
        during:
        cooldownArrDepLeft = cooldownArrDepLeft - int32(1);
      state DEPARTURE_BURN
        entry:
        burnActive = true;
        during:
        controlAcc = dvCmd / tBurn;
        stepsLeft = stepsLeft - int32(1);
        exit:
        dvDepLog = zeros(3,1);
      (default) -> ARRIVAL_BURN
      ARRIVAL_BURN -> INTER_BURN_COOLDOWN : [stepsArrLeft <= int32(0)]
          | {cooldownArrDepLeft = nCooldownArrDep;
          | dvArrLog = zeros(3,1);}
      INTER_BURN_COOLDOWN -> DEPARTURE_BURN : [cooldownArrDepLeft <= int32(0)]
          | {dvCmd_gl = guidanceLaw(SCPosition, SCVelocity, k);
          | rPred = propagateState(SCPosition, SCVelocity + dvCmd_gl, WP_dtArc, []);
          | kNext = mod(k, WP_NWaypoints) + int32(1);
          | rTarget = WP_waypointPosition(kNext,:)';
          | err = rTarget - rPred;
          | Phi_rv = WP_STMArcs(1:3, 4:6, k);
          | dvCmd = dvCmd_gl + inv(Phi_rv) * err;
          | dvDepLog = dvCmd;}
    state NO_BURN
      entry:
      controlAcc = zeros(3,1);
      stepsLeft = int32(0);
      currentWpIdx = k;
    (default) -> (junction 56)
    (junction 56) -> SINGLE_BURN [order 1] : [WP_burnStrategy == burnStrategyVariant.SINGLE]
        |
        | {dvCmd_gl = guidanceLaw(SCPosition, SCVelocity, k);
        | [rPred, rTraj] = propagateState(SCPosition, SCVelocity + dvCmd_gl, WP_dtArc, []);
        | kNext = mod(k, WP_NWaypoints) + int32(1);
        | rTarget = WP_waypointPosition(kNext,:)';
        | err = rTarget - rPred;
        | Phi_rv = WP_STMArcs(1:3, 4:6, k);
        | dvCmd = dvCmd_gl + inv(Phi_rv) * err;
        | }
    (junction 56) -> (junction 61) [order 2]
    (junction 61) -> TWO_STAGE [order 1] : [WP_burnStrategy == burnStrategyVariant.TWO_STAGE]
        |
        | {dvArr = WP_waypointVelocity(k, :)' - SCVelocity;
        |  dvArrLog = dvArr;
        |  stepsArrLeft = int32(nSteps);}
    (junction 61) -> NO_BURN [order 2]
  state INIT
    entry:
    nSteps = int32(tBurn/dtSim);
    nCooldownArrDep = int32(1.0/dtSim);
  state IDLE
    entry:
    controlAcc = zeros(3,1);
    burnActive = false;
    currentWpIdx = k;
    during:
    currentWpIdx = k;
  state res = nearWaypoint(SCPosition, k) [function]
  state dvCmd = guidanceLaw(SCPosition,SCVelocity,k) [function]
  state COOLDOWN
    entry:
    controlAcc = zeros(3,1);
    burnActive = false;
    during:
    cooldownLeft = cooldownLeft - int32(1);
    currentWpIdx = k;
  state gravAttraction = gravAccel(SCPosition) [function]
  IDLE -> ACTIVE_BURN : [nearWaypoint(SCPosition, k)]
      | {stepsLeft = nSteps; }
  (default) -> INIT
  INIT -> IDLE
  COOLDOWN -> IDLE : [cooldownLeft <= int32(0)]
  ACTIVE_BURN -> COOLDOWN : [stepsLeft <= int32(0)]
      |
      | {k = mod(k, WP_NWaypoints) + int32(1);
      | [~, rTraj2, dt_new] = propagateState(SCPosition, SCVelocity, ...
      | WP_dtArc, WP_waypointPosition(k,:));
      | cooldownLeft = int32(dt_new / dtSim);}
  data: SCPosition function_input double size=3; k function_input int32 size=1; res function_output; SCPosition function_input double size=3; SCVelocity function_input double size=3; k function_input int32 size=1; dvCmd function_output; SCPosition function_input double size=3; gravAttraction function_output; rF function_output; r0 function_input; v0 function_input; dt_arc function_input; asteroidAngularVelocity parameter; rr function_output; wp_r function_input; dt_upd function_output double; WP_NWaypoints parameter; dtSim input; currentWpIdx output; controlAcc output; burnActive output; k local int32 size=1 =1; tBurn input; nSteps local int32 size=1 =0; stepsLeft local int32 size=1 =0; SCPosition input size=3; SCVelocity input; cooldownLeft local int32 size=1 =0; WP_dtArc parameter; WP_burnStrategy parameter; WP_waypointVelocity parameter; dvArr local double size=[3 1] =[0; 0; 0]; stepsArrLeft local int32 size=1 =0; dvArrLog output; dvDepLog output; nCooldownArrDep local int32 size=1 =0; cooldownArrDepLeft local int32 size=1 =0; WP_STMArcs parameter; WP_waypointPosition parameter; Phi_rv local double size=[3 3] =eye(3); err local double size=3 =[0;0;0]; kNext local int32 size=1 =2; rPred local double size=3 =[0;0;0]; rTarget local double size=3 =[0;0;0]; rTraj output; dvCmd output double size=[3 1] =[0;0;0]; rTraj2 output double size=[100 3] =zeros(100, 3); dvCmd_gl local double size=3 =[0;0;0]; dt_new output double size=1 =0
  function [rF, rr, dt_upd] = propagateState(r0, v0, dt_arc, wp_r):
    | function [rF, rr, dt_upd] = propagateState(r0, v0, dt_arc, wp_r)
    | 
    |     %#codegen
    |     % State propagation using Runge-Kutta 4
    | 
    |     nStepsRK = 100;
    |     h = dt_arc / nStepsRK;    % step-size
    |     propagatedPos = r0;
    |     propagatedVel = v0;
    |     rr = zeros(nStepsRK, 3);
    | 
    |     dt_upd = dt_arc;
    |     distMin = Inf;
    |     if ~isempty(wp_r)
    |         updateDt = true;
    |     else
    |         updateDt = false;
    |     end
    | 
    |     for ii = 1:nStepsRK
    |         % Function at ii-1 
    |         g_old = gravAccel(propagatedPos);
    |         fr_old = propagatedVel;
    |         fv_old = g_old - 2*cross(asteroidAngularVelocity, propagatedVel) - cross(asteroidAngularVelocity, cross(asteroidAngularVelocity, propagatedPos));
    | 
    |         % First predictor P1
    |         r_P1 = propagatedPos + 0.5*h*fr_old;
    |         v_P1 = propagatedVel + 0.5*h*fv_old;
    |         g_P1 = gravAccel(r_P1);
    |         fr_P1 = v_P1;
    |         fv_P1 = g_P1 - 2*cross(asteroidAngularVelocity, v_P1) - cross(asteroidAngularVelocity, cross(asteroidAngularVelocity, r_P1));
    | 
    |         % Second predictor P2
    |         r_P2 = propagatedPos + 0.5*h*fr_P1;
    |         v_P2 = propagatedVel + 0.5*h*fv_P1;
    |         g_P2 = gravAccel(r_P2);
    |         fr_P2 = v_P2;
    |         fv_P2 = g_P2 - 2*cross(asteroidAngularVelocity, v_P2) - cross(asteroidAngularVelocity, cross(asteroidAngularVelocity, r_P2));
    | 
    |         % Third predictor P3
    |         r_P3 = propagatedPos + h*fr_P2;
    |         v_P3 = propagatedVel + h*fv_P2;
    |         g_P3 = gravAccel(r_P3);
    |         fr_P3 = v_P3;
    |         fv_P3 = g_P3 - 2*cross(asteroidAngularVelocity, v_P3) - cross(asteroidAngularVelocity, cross(asteroidAngularVelocity, r_P3));
    | 
    |         % Corrector
    |         propagatedPos = propagatedPos + h/6 * (fr_old + 2*fr_P1 + 2*fr_P2 + fr_P3);
    |         propagatedVel = propagatedVel + h/6 * (fv_old + 2*fv_P1 + 2*fv_P2 + fv_P3);
    | 
    |         % Save for debug
    |         rr(ii, :) = propagatedPos;
    | 
    |         % Update dt if necessary
    |         if updateDt
    |             dist = norm(propagatedPos - wp_r');
    |             if dist < distMin
    |                 distMin = dist;
    |             else
    |                 dt_upd = ii*h;
    |                 break
    |             end
    |         end
    |     end
    | 
    |     rF = propagatedPos;
    | 
    | end

== matlab function ARIES/Attitude Control/Attitude error DCM copy/MATLAB Function ==
  data: Ae_vec output; Ce input
function Ae_vec = AttErrVec(Ce)
    %#codegen

    if trace(Ce) < -0.5
        % Extract rotation axis
        CeI = Ce + eye(3);
        [~, idx] = max(diag(CeI)); % Find largest diagonal element
        n = CeI(:, idx);
        n = n / norm(n);
        if n(idx) < 0
            n = -n;
        end
        Ae_vec = pi*n;
    else
        Ae = Ce - Ce';
        Ae_vec = [Ae(3,2); Ae(1,3); Ae(2,1)];
    end

end
